simulink model "lab_otu_pid"  (R2022a)
settings: Solver=VariableStepAuto  StartTime=0.0  StopTime=10.0  RelTol=1e-3
settings Model: Creator=salgi  LastModifiedBy=salgi

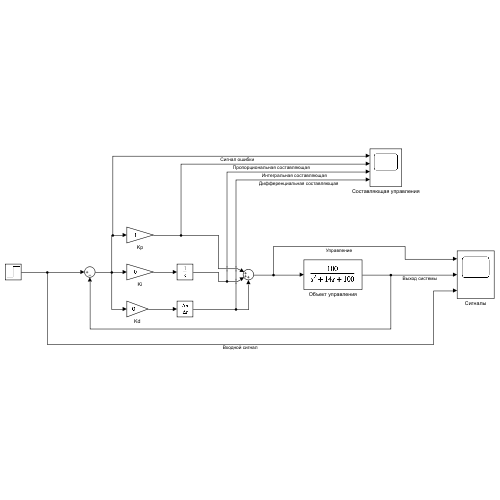
[thumbnail: Simulink's stored preview of the top-level diagram]
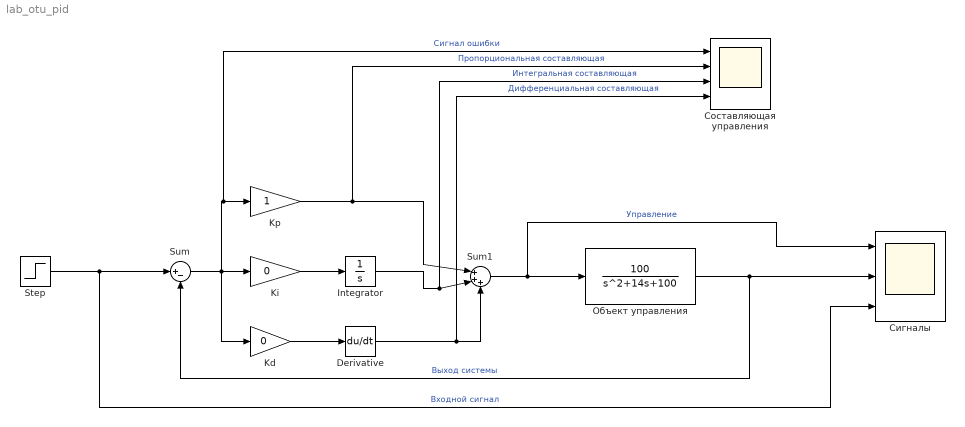
== system lab_otu_pid ==
  Derivative : Derivative
  Integrator : Integrator
  Kd : Gain  Gain=0
  Ki : Gain  Gain=0
  Kp : Gain
  Step : Step  SampleTime=0
  Sum : Sum  Inputs=|+-
  Sum1 : Sum  Inputs=|+++  RndMeth=Nearest
  Объект управления : TransferFcn  Numerator=[100]  Denominator=[1 14 100]
  Сигналы : Scope  NumInputPorts=3
  Составляющая управления : Scope  NumInputPorts=4
  wires:
  Step/1 -> Sum/1, Сигналы/3  "Входной сигнал"
  Sum/1 -> Составляющая управления/1, Kp/1, Kd/1, Ki/1  "Сигнал ошибки"
  Ki/1 -> Integrator/1
  Kd/1 -> Derivative/1
  Kp/1 -> Составляющая управления/2, Sum1/1  "Пропорциональная составляющая"
  Integrator/1 -> Составляющая управления/3, Sum1/2  "Интегральная составляющая"
  Derivative/1 -> Составляющая управления/4, Sum1/3  "Дифференциальная составляющая"
  Sum1/1 -> Сигналы/1, Объект управления/1  "Управление"
  Объект управления/1 -> Sum/2, Сигналы/2  "Выход системы"
